simulink model "V0"  (R2026b)
settings: Solver=VariableStepAuto  MaxStep=1e-3
undefined symbols (not defined in the file): X, Y, Z
libraries: sm_lib x30, nesl_utility x7
settings Model: Creator=Alex  LastModifiedBy=Providenta
settings RTWCC: GPUComputeCapability=5.0
settings SimscapeCC: SimscapeUseEnergyAccounting=off
settings ExplorerConfigSet: InternalSimMechanicsExplorerSettings=|
  | <ExplorerConfiguration>
  | 
  |   <canonicalview>default</canonicalview>
  | 
  |   <TilePanel>
  |     <TileInfo>
  |       <Tiles Columns="1" Count="1" Height="506" Rows="1" Width="626">
  |         <Row Weight="1"/>
  |         <Column Weight="1"/>
  |         <Tile Height="1" Width="1" X="0" Y="0"/>
  |       </Tiles>
  |     </TileInfo>
  |     <SceneInfo>
  |       <SceneViewer>
  |         <IsThisViewStd>
  |           <IsStandardView>off</IsStandardView>
  |           <StandardViewName>Front</StandardViewName>
  |         </IsThisViewStd>
  |         <BGColor>
  |           <R>1</R>
  |           <G>1</G>
  |           <B>1</B>
  |           <A>1</A>
  |         </BGColor>
  |         <Camera>
  |           <DoPerspective>off</DoPerspective>
  |           <Position>
  |             <X>-1.2632471406802588</X>
  |             <Y>1.7763638648148106</Y>
  |             <Z>1.5649874221387672</Z>
  |           </Position>
  |           <Center>
  |             <X>0.25024160266871465</X>
  |             <Y>0.26287512146583708</Y>
  |             <Z>0.051498678789793695</Z>
  |           </Center>
  |           <Up>
  |             <X>0.40824829046386307</X>
  |             <Y>-0.40824829046386307</Y>
  |             <Z>0.81649658092772615</Z>
  |           </Up>
  |           <XLim>0.3536848912827506</XLim>
  |           <YLim>0.3536848912827506</YLim>
  |           <ViewLimDist>0.01</ViewLimDist>
  |         </Camera>
  |       </SceneViewer>
  |     </SceneInfo>
  |   </TilePanel>
  | 
  |   <MechEditorPanel>
  |     <GfxPanelCameraMap/>
  |     <Cameras/>
  |     <VideoCreator>
  |       <IncludeTiles>All</IncludeTiles>
  |       <IncludeTime>on</IncludeTime>
  |       <IncludeWorldFrame>off</IncludeWorldFrame>
  |       <PlaybackSpeedRatio>1</PlaybackSpeedRatio>
  |       <FrameRate>30</FrameRate>
  |       <FrameSize>auto</FrameSize>
  |       <VideoFormat>UncompressedAVI</VideoFormat>
  |     </VideoCreator>
  |   </MechEditorPanel>
  | 
  |   <PlaybackSettings>
  |     <PlaybackSpeedFactor>2</PlaybackSpeedFactor>
  |   </PlaybackSettings>
  | 
  | </ExplorerConfiguration>

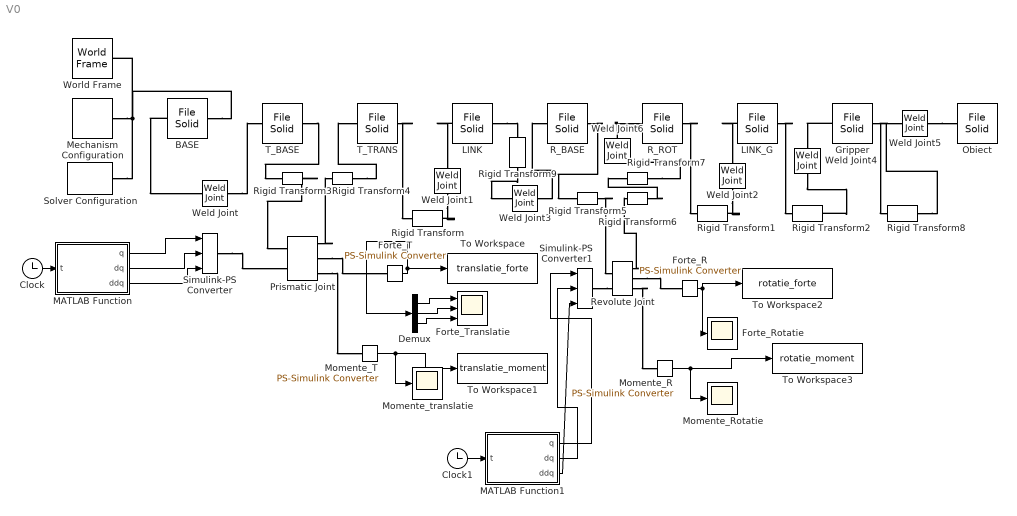
== system V0 ==
  BASE : sm_lib/Body Elements/File Solid  ExtGeomFileName=C:\Users\Georgian\Documents\PROBO\Objects\Links\Base.CATPart  UnitType=FromFile  ExtGeomFileUnits=m  StepReaderType=HEX  ExportConvexHullGeometry=off  InertiaType=CalculateFromGeometry  BasedOnType=DensityFromFile  Density=1000  DensityUnits=kg/m^3  Mass=1  MassUnits=kg  CenterOfMass=[0 0 0]  CenterOfMassUnits=m  MomentsOfInertia=[1 1 1]  MomentsOfInertiaUnits=kg*m^2  ProductsOfInertia=[0 0 0]  ProductsOfInertiaUnits=kg*m^2  GraphicType=FromGeometry  MarkerShape=Sphere  MarkerSize=10  GraphicVisPropType=SimpleVisualProperties  GraphicDiffuseColor=[0.5 0.5 0.5]  GraphicOpacity=1  GraphicSpecularColor=[0.5 0.5 0.5 1.0]  GraphicAmbientColor=[0.15 0.15 0.15 1.0]  GraphicEmissiveColor=[0.0 0.0 0.0 1.0]  GraphicShininess=75  DoExposeReferenceFrame=on  SerializedFrames=<Frames><Frame><Id>Frame1</Id><Value><Name>Main_LINK</Name><Origin><Source>GeometricFeature</Source><FeatureName>planar surface 2</FeatureName></Origin><PrimaryAxis><DefinedDirection>+Y</DefinedDirection><Source>ReferenceFrame</Source><SourceDirection>-Y</SourceDirection><FeatureName></FeatureName></PrimaryAxis><SecondaryAxis><DefinedDirection>+X</DefinedDirection><Source>ReferenceFrame</Source><SourceDirection>+X</SourceDirection><FeatureName></FeatureName></SecondaryAxis></Value></Frame></Frames>
  Clock : Clock
  Clock1 : Clock
  Demux : Demux  Outputs=3
  Forte_R : nesl_utility/PS-Simulink Converter  PhysicalDomain=network_engine_domain  SubClassName=ps_output  LeftPortType=input  RightPortType=output  PseudoPeriodic=off  Frequencies=[]  VectorFormat=inherit  Unit=inherit  AffineConversion=off
  Forte_Rotatie : Scope
      settings: ActiveDisplayYMinimum=-165.96901704363273  ActiveDisplayYMaximum=591.60143737609849  DataLoggingVariableName=ScopeData2
  Forte_T : nesl_utility/PS-Simulink Converter  PhysicalDomain=network_engine_domain  SubClassName=ps_output  LeftPortType=input  RightPortType=output  PseudoPeriodic=off  Frequencies=[]  VectorFormat=inherit  Unit=inherit  AffineConversion=off
  Forte_Translatie : Scope  NumInputPorts=3
      settings: ActiveDisplayYMinimum=-453.2641950281286  ActiveDisplayYMaximum=842.77836421107531
  Gripper : sm_lib/Body Elements/File Solid  ExtGeomFileName=C:\Users\Georgian\Documents\PROBO\Objects\Subansamblu_Gripper_fara_ob.stp  UnitType=FromFile  ExtGeomFileUnits=m  StepReaderType=HEX  ExportConvexHullGeometry=off  InertiaType=Custom  BasedOnType=DensityFromFile  Density=1000  DensityUnits=kg/m^3  Mass=4.055  MassUnits=kg  CenterOfMass=[0.0003906 79.531 -4.359]  CenterOfMassUnits=mm  MomentsOfInertia=[0.036 0.027 0.02]  MomentsOfInertiaUnits=kg*m^2  ProductsOfInertia=[-1.269e-5 -0.002 -1.039e-8]  ProductsOfInertiaUnits=kg*m^2  GraphicType=FromGeometry  MarkerShape=Sphere  MarkerSize=10  GraphicVisPropType=SimpleVisualProperties  GraphicDiffuseColor=[0.5 0.5 0.5]  GraphicOpacity=1  GraphicSpecularColor=[0.5 0.5 0.5 1.0]  GraphicAmbientColor=[0.15 0.15 0.15 1.0]  GraphicEmissiveColor=[0.0 0.0 0.0 1.0]  GraphicShininess=75  DoExposeReferenceFrame=off  SerializedFrames=<Frames><Frame><Id>Frame1</Id><Value><Name>R</Name><Origin><Source>GeometricFeature</Source><FeatureName>planar surface 481</FeatureName></Origin><PrimaryAxis><DefinedDirection>+Y</DefinedDirection><Source>ReferenceFrame</Source><SourceDirection>+Y</SourceDirection><FeatureName></FeatureName></PrimaryAxis><SecondaryAxis><DefinedDirection>+X</DefinedDirection><Source>ReferenceFrame</Source><SourceDirection>+X</SourceDirection><FeatureName></FeatureName></SecondaryAxis></Value></Frame><Frame><Id>Frame2</Id><Value><Name>F</Name><Origin><Source>GeometricFeature</Source><FeatureName>planar surface 1100</FeatureName></Origin><PrimaryAxis><DefinedDirection>+Z</DefinedDirection><Source>ReferenceFrame</Source><SourceDirection>+Z</SourceDirection><FeatureName></FeatureName></PrimaryAxis><SecondaryAxis><DefinedDirection>+X</DefinedDirection><Source>ReferenceFrame</Source><SourceDirection>+X</SourceDirection><FeatureName></FeatureName></SecondaryAxis></Value></Frame></Frames>
  LINK : sm_lib/Body Elements/File Solid  ExtGeomFileName=C:\Users\Georgian\Documents\PROBO\Objects\Links\Cot.CATPart  UnitType=FromFile  ExtGeomFileUnits=m  StepReaderType=HEX  ExportConvexHullGeometry=off  InertiaType=CalculateFromGeometry  BasedOnType=DensityFromFile  Density=1000  DensityUnits=kg/m^3  Mass=1  MassUnits=kg  CenterOfMass=[0 0 0]  CenterOfMassUnits=m  MomentsOfInertia=[1 1 1]  MomentsOfInertiaUnits=kg*m^2  ProductsOfInertia=[0 0 0]  ProductsOfInertiaUnits=kg*m^2  GraphicType=FromGeometry  MarkerShape=Sphere  MarkerSize=10  GraphicVisPropType=SimpleVisualProperties  GraphicDiffuseColor=[0.5 0.5 0.5]  GraphicOpacity=1  GraphicSpecularColor=[0.5 0.5 0.5 1.0]  GraphicAmbientColor=[0.15 0.15 0.15 1.0]  GraphicEmissiveColor=[0.0 0.0 0.0 1.0]  GraphicShininess=75  DoExposeReferenceFrame=off  SerializedFrames=|
      | <Frames>
      | 
      |   <Frame>
      |     <Id>Frame1</Id>
      |     <Value>
      |       <Name>F1</Name>
      |       <Origin>
      |         <Source>GeometricFeature</Source>
      |         <FeatureName>planar surface 2</FeatureName>
      |       </Origin>
      |       <PrimaryAxis>
      |         <DefinedDirection>+Z</DefinedDirection>
      |         <Source>ReferenceFrame</Source>
      |         <SourceDirection>+Z</SourceDirection>
      |         <FeatureName></FeatureName>
      |       </PrimaryAxis>
      |       <SecondaryAxis>
      |         <DefinedDirection>+X</DefinedDirection>
      |         <Source>ReferenceFrame</Source>
      |         <SourceDirection>+X</SourceDirection>
      |         <FeatureName></FeatureName>
      |       </SecondaryAxis>
      |     </Value>
      |   </Frame>
      | 
      |   <Frame>
      |     <Id>Frame2</Id>
      |     <Value>
      |       <Name>F2</Name>
      |       <Origin>
      |         <Source>GeometricFeature</Source>
      |         <FeatureName>planar surface 4</FeatureName>
      |       </Origin>
      |       <PrimaryAxis>
      |         <DefinedDirection>+Z</DefinedDirection>
      |         <Source>ReferenceFrame</Source>
      |         <SourceDirection>+Z</SourceDirection>
      |         <FeatureName></FeatureName>
      |       </PrimaryAxis>
      |       <SecondaryAxis>
      |         <DefinedDirection>+X</DefinedDirection>
      |         <Source>ReferenceFrame</Source>
      |         <SourceDirection>+X</SourceDirection>
      |         <FeatureName></FeatureName>
      |       </SecondaryAxis>
      |     </Value>
      |   </Frame>
      | 
      | </Frames>
  LINK_G : sm_lib/Body Elements/File Solid  ExtGeomFileName=C:\Users\Georgian\Documents\PROBO\Objects\LINK_MODUL2\LINK_G_MR.step  UnitType=FromFile  ExtGeomFileUnits=m  StepReaderType=HEX  ExportConvexHullGeometry=off  InertiaType=Custom  BasedOnType=DensityFromFile  Density=1000  DensityUnits=kg/m^3  Mass=1.753  MassUnits=kg  CenterOfMass=[0 -38.58 157.13]  CenterOfMassUnits=mm  MomentsOfInertia=[0.011 0.013 0.001]  MomentsOfInertiaUnits=kg*m^2  ProductsOfInertia=[0 0 0.001]  ProductsOfInertiaUnits=kg*m^2  GraphicType=FromGeometry  MarkerShape=Sphere  MarkerSize=10  GraphicVisPropType=SimpleVisualProperties  GraphicDiffuseColor=[0.5 0.5 0.5]  GraphicOpacity=1  GraphicSpecularColor=[0.5 0.5 0.5 1.0]  GraphicAmbientColor=[0.15 0.15 0.15 1.0]  GraphicEmissiveColor=[0.0 0.0 0.0 1.0]  GraphicShininess=75  DoExposeReferenceFrame=off  SerializedFrames=<Frames><Frame><Id>Frame1</Id><Value><Name>R</Name><Origin><Source>GeometricFeature</Source><FeatureName>planar surface 1</FeatureName></Origin><PrimaryAxis><DefinedDirection>+Z</DefinedDirection><Source>ReferenceFrame</Source><SourceDirection>+Z</SourceDirection><FeatureName></FeatureName></PrimaryAxis><SecondaryAxis><DefinedDirection>+X</DefinedDirection><Source>ReferenceFrame</Source><SourceDirection>+X</SourceDirection><FeatureName></FeatureName></SecondaryAxis></Value></Frame><Frame><Id>Frame2</Id><Value><Name>F</Name><Origin><Source>GeometricFeature</Source><FeatureName>planar surface 41</FeatureName></Origin><PrimaryAxis><DefinedDirection>+Y</DefinedDirection><Source>ReferenceFrame</Source><SourceDirection>+Y</SourceDirection><FeatureName></FeatureName></PrimaryAxis><SecondaryAxis><DefinedDirection>+X</DefinedDirection><Source>ReferenceFrame</Source><SourceDirection>+X</SourceDirection><FeatureName></FeatureName></SecondaryAxis></Value></Frame></Frames>
  MATLAB Function : MATLAB Function  TreatAsAtomicUnit=on
  MATLAB Function1 : MATLAB Function  TreatAsAtomicUnit=on
  Mechanism Configuration : sm_lib/Utilities/Mechanism Configuration  UniformGravity=Constant  GravityVector=[0 0 -9.80665]  GravityVectorUnits=m/s^2  LinearizationDelta=0.001  JointModeTransitionNonlinearIterations=2
  Momente_R : nesl_utility/PS-Simulink Converter  PhysicalDomain=network_engine_domain  SubClassName=ps_output  LeftPortType=input  RightPortType=output  PseudoPeriodic=off  Frequencies=[]  VectorFormat=inherit  Unit=inherit  AffineConversion=off
  Momente_Rotatie : Scope
      settings: ActiveDisplayYMinimum=-181.02759056182146  ActiveDisplayYMaximum=207.23761817348006  DataLoggingVariableName=ScopeData3
  Momente_T : nesl_utility/PS-Simulink Converter  PhysicalDomain=network_engine_domain  SubClassName=ps_output  LeftPortType=input  RightPortType=output  PseudoPeriodic=off  Frequencies=[]  VectorFormat=inherit  Unit=inherit  AffineConversion=off
  Momente_translatie : Scope
      settings: ActiveDisplayYMinimum=-251.95677444746502  ActiveDisplayYMaximum=342.42507637342931
  Obiect : sm_lib/Body Elements/File Solid  ExtGeomFileName=C:\Users\Georgian\Documents\PROBO\Objects\Paralelipiped.CATPart  UnitType=FromFile  ExtGeomFileUnits=m  StepReaderType=HEX  ExportConvexHullGeometry=off  InertiaType=Custom  BasedOnType=DensityFromFile  Density=1000  DensityUnits=kg/m^3  Mass=32.54  MassUnits=kg  CenterOfMass=[0 0 115]  CenterOfMassUnits=mm  MomentsOfInertia=[0.171 0.231 0.115]  MomentsOfInertiaUnits=kg*m^2  ProductsOfInertia=[0 0 0]  ProductsOfInertiaUnits=kg*m^2  GraphicType=FromGeometry  MarkerShape=Sphere  MarkerSize=10  GraphicVisPropType=SimpleVisualProperties  GraphicDiffuseColor=[0.5 0.5 0.5]  GraphicOpacity=1  GraphicSpecularColor=[0.5 0.5 0.5 1.0]  GraphicAmbientColor=[0.15 0.15 0.15 1.0]  GraphicEmissiveColor=[0.0 0.0 0.0 1.0]  GraphicShininess=75  DoExposeReferenceFrame=off  SerializedFrames=<Frames><Frame><Id>Frame1</Id><Value><Name>R</Name><Origin><Source>GeometricFeature</Source><FeatureName>planar surface 4</FeatureName></Origin><PrimaryAxis><DefinedDirection>+Z</DefinedDirection><Source>ReferenceFrame</Source><SourceDirection>+Z</SourceDirection><FeatureName></FeatureName></PrimaryAxis><SecondaryAxis><DefinedDirection>+X</DefinedDirection><Source>ReferenceFrame</Source><SourceDirection>+X</SourceDirection><FeatureName></FeatureName></SecondaryAxis></Value></Frame></Frames>
  Prismatic Joint : sm_lib/Joints/Prismatic Joint  JointMode=Normal  CompositeWrenchDir=FollowerOnBase  CompositeWrenchFrame=BaseFrame  SenseConstraintForce=off  SenseConstraintTorque=off  SenseTotalForce=on  SenseTotalTorque=on  PositionTargetSpecify=off  PositionTargetPriority=High  PositionTargetValue=0  PositionTargetValueUnits=m  VelocityTargetSpecify=off  VelocityTargetPriority=High  VelocityTargetValue=0  VelocityTargetValueUnits=m/s  EquilibriumPosition=0  EquilibriumPositionUnits=m  SpringStiffness=0  SpringStiffnessUnits=N/m  DampingCoefficient=0  DampingCoefficientUnits=N/(m/s)  LowerLimitSpecify=off  LowerLimitBound=-1  LowerLimitBoundUnits=m  LowerLimitStiffness=1e6  LowerLimitStiffnessUnits=N/m  LowerLimitDamping=1e3  LowerLimitDampingUnits=N/(m/s)  LowerLimitTransitionRegionWidth=1e-4  LowerLimitTransitionRegionWidthUnits=m  UpperLimitSpecify=off  UpperLimitBound=1  UpperLimitBoundUnits=m  UpperLimitStiffness=1e6  UpperLimitStiffnessUnits=N/m  UpperLimitDamping=1e3  UpperLimitDampingUnits=N/(m/s)  UpperLimitTransitionRegionWidth=1e-4  UpperLimitTransitionRegionWidthUnits=m  TorqueActuationMode=ComputedTorque  MotionActuationMode=InputMotion  SensePosition=off  SenseVelocity=off  SenseAcceleration=off  SenseTorqueForce=off  SenseLowerLimitTorqueForce=off  SenseUpperLimitTorqueForce=off
  R_BASE : sm_lib/Body Elements/File Solid  ExtGeomFileName=C:\Users\Georgian\Documents\PROBO\Objects\MODUL 2\R_STABIL\R_STABIL.stp  UnitType=FromFile  ExtGeomFileUnits=m  StepReaderType=HEX  ExportConvexHullGeometry=off  InertiaType=Custom  BasedOnType=DensityFromFile  Density=1000  DensityUnits=kg/m^3  Mass=4.576  MassUnits=kg  CenterOfMass=[0 0 -42.1]  CenterOfMassUnits=mm  MomentsOfInertia=[3.787e-2 3.787e-2 8.59e-3]  MomentsOfInertiaUnits=kg*m^2  ProductsOfInertia=[0 0 0]  ProductsOfInertiaUnits=kg*m^2  GraphicType=FromGeometry  MarkerShape=Sphere  MarkerSize=10  GraphicVisPropType=SimpleVisualProperties  GraphicDiffuseColor=[0.5 0.5 0.5]  GraphicOpacity=1  GraphicSpecularColor=[0.5 0.5 0.5 1.0]  GraphicAmbientColor=[0.15 0.15 0.15 1.0]  GraphicEmissiveColor=[0.0 0.0 0.0 1.0]  GraphicShininess=75  DoExposeReferenceFrame=off  SerializedFrames=<Frames><Frame><Id>Frame1</Id><Value><Name>R</Name><Origin><Source>GeometricFeature</Source><FeatureName>planar surface 141</FeatureName></Origin><PrimaryAxis><DefinedDirection>+Z</DefinedDirection><Source>ReferenceFrame</Source><SourceDirection>+Z</SourceDirection><FeatureName></FeatureName></PrimaryAxis><SecondaryAxis><DefinedDirection>+X</DefinedDirection><Source>ReferenceFrame</Source><SourceDirection>+X</SourceDirection><FeatureName></FeatureName></SecondaryAxis></Value></Frame><Frame><Id>Frame2</Id><Value><Name>F2</Name><Origin><Source>GeometricFeature</Source><FeatureName>planar surface 199</FeatureName></Origin><PrimaryAxis><DefinedDirection>+Z</DefinedDirection><Source>ReferenceFrame</Source><SourceDirection>+Z</SourceDirection><FeatureName></FeatureName></PrimaryAxis><SecondaryAxis><DefinedDirection>+X</DefinedDirection><Source>ReferenceFrame</Source><SourceDirection>+X</SourceDirection><FeatureName></FeatureName></SecondaryAxis></Value></Frame></Frames>
  R_ROT : sm_lib/Body Elements/File Solid  ExtGeomFileName=C:\Users\Georgian\Documents\PROBO\Objects\MODUL 2\R_MOBIL\R_MOBIL.stp  UnitType=FromFile  ExtGeomFileUnits=m  StepReaderType=HEX  ExportConvexHullGeometry=off  InertiaType=Custom  BasedOnType=DensityFromFile  Density=1000  DensityUnits=kg/m^3  Mass=0.3668  MassUnits=kg  CenterOfMass=[0 0 56.03]  CenterOfMassUnits=mm  MomentsOfInertia=[1.086e-4 1.069e-4 1.647e-4]  MomentsOfInertiaUnits=kg*m^2  ProductsOfInertia=[0 0 -2.83e-7]  ProductsOfInertiaUnits=kg*m^2  GraphicType=FromGeometry  MarkerShape=Sphere  MarkerSize=10  GraphicVisPropType=SimpleVisualProperties  GraphicDiffuseColor=[0.5 0.5 0.5]  GraphicOpacity=1  GraphicSpecularColor=[0.5 0.5 0.5 1.0]  GraphicAmbientColor=[0.15 0.15 0.15 1.0]  GraphicEmissiveColor=[0.0 0.0 0.0 1.0]  GraphicShininess=75  DoExposeReferenceFrame=off  SerializedFrames=<Frames><Frame><Id>Frame1</Id><Value><Name>R</Name><Origin><Source>GeometricFeature</Source><FeatureName>planar surface 20</FeatureName></Origin><PrimaryAxis><DefinedDirection>+Y</DefinedDirection><Source>ReferenceFrame</Source><SourceDirection>+Y</SourceDirection><FeatureName></FeatureName></PrimaryAxis><SecondaryAxis><DefinedDirection>+X</DefinedDirection><Source>ReferenceFrame</Source><SourceDirection>+X</SourceDirection><FeatureName></FeatureName></SecondaryAxis></Value></Frame><Frame><Id>Frame2</Id><Value><Name>F</Name><Origin><Source>GeometricFeature</Source><FeatureName>planar surface 22</FeatureName></Origin><PrimaryAxis><DefinedDirection>+Z</DefinedDirection><Source>ReferenceFrame</Source><SourceDirection>+Z</SourceDirection><FeatureName></FeatureName></PrimaryAxis><SecondaryAxis><DefinedDirection>+X</DefinedDirection><Source>ReferenceFrame</Source><SourceDirection>+X</SourceDirection><FeatureName></FeatureName></SecondaryAxis></Value></Frame></Frames>
  Revolute Joint : sm_lib/Joints/Revolute Joint  JointMode=Normal  CompositeWrenchDir=FollowerOnBase  CompositeWrenchFrame=BaseFrame  SenseConstraintForce=off  SenseConstraintTorque=off  SenseTotalForce=on  SenseTotalTorque=on  PositionTargetSpecify=off  PositionTargetPriority=High  PositionTargetValue=0  PositionTargetValueUnits=deg  VelocityTargetSpecify=off  VelocityTargetPriority=High  VelocityTargetValue=0  VelocityTargetValueUnits=deg/s  EquilibriumPosition=0  EquilibriumPositionUnits=deg  SpringStiffness=0  SpringStiffnessUnits=N*m/deg  DampingCoefficient=0  DampingCoefficientUnits=N*m/(deg/s)  LowerLimitSpecify=off  LowerLimitBound=-90  LowerLimitBoundUnits=deg  LowerLimitStiffness=1e4  LowerLimitStiffnessUnits=N*m/deg  LowerLimitDamping=10  LowerLimitDampingUnits=N*m/(deg/s)  LowerLimitTransitionRegionWidth=0.1  LowerLimitTransitionRegionWidthUnits=deg  UpperLimitSpecify=off  UpperLimitBound=90  UpperLimitBoundUnits=deg  UpperLimitStiffness=1e4  UpperLimitStiffnessUnits=N*m/deg  UpperLimitDamping=10  UpperLimitDampingUnits=N*m/(deg/s)  UpperLimitTransitionRegionWidth=0.1  UpperLimitTransitionRegionWidthUnits=deg  TorqueActuationMode=ComputedTorque  MotionActuationMode=InputMotion  SensePosition=off  SenseVelocity=off  SenseAcceleration=off  SenseTorqueForce=off  SenseLowerLimitTorqueForce=off  SenseUpperLimitTorqueForce=off
  Rigid Transform : sm_lib/Frames and Transforms/Rigid Transform  RotationMethod=RotationSequence  FollAlignAxisA=+X  BaseAlignAxisA=+Y  FollAlignAxisB=+Y  BaseAlignAxisB=+Z  RotationStandardAxis=+Y  RotationAngle=90  RotationAngleUnits=deg  RotationArbitraryAxis=[0 0 1]  RotationSequenceAxes=FollowerAxes  RotationSequence=YZX  RotationSequenceAngles=[90 180 0]  RotationSequenceAnglesUnits=deg  RotationMatrix=[1 0 0;0 1 0;0 0 1]  Quaternion=[1 0 0 0]  TranslationMethod=None  TranslationCartesianOffset=[0 0 0]  TranslationCartesianOffsetUnits=m  TranslationStandardAxis=+Z  TranslationStandardOffset=0  TranslationStandardOffsetUnits=m  TranslationROffset=0  TranslationROffsetUnits=m  TranslationThetaOffset=0  TranslationThetaOffsetUnits=deg  TranslationZOffset=0  TranslationZOffsetUnits=m
  Rigid Transform1 : sm_lib/Frames and Transforms/Rigid Transform  RotationMethod=RotationSequence  FollAlignAxisA=+X  BaseAlignAxisA=+Y  FollAlignAxisB=+Y  BaseAlignAxisB=+Z  RotationStandardAxis=+Z  RotationAngle=180  RotationAngleUnits=deg  RotationArbitraryAxis=[0 0 1]  RotationSequenceAxes=FollowerAxes  RotationSequence=ZXY  RotationSequenceAngles=[180 0 0]  RotationSequenceAnglesUnits=deg  RotationMatrix=[1 0 0;0 1 0;0 0 1]  Quaternion=[1 0 0 0]  TranslationMethod=Cartesian  TranslationCartesianOffset=[0 20 0]  TranslationCartesianOffsetUnits=mm  TranslationStandardAxis=+Z  TranslationStandardOffset=0  TranslationStandardOffsetUnits=m  TranslationROffset=0  TranslationROffsetUnits=m  TranslationThetaOffset=0  TranslationThetaOffsetUnits=deg  TranslationZOffset=0  TranslationZOffsetUnits=m
  Rigid Transform2 : sm_lib/Frames and Transforms/Rigid Transform  RotationMethod=RotationSequence  FollAlignAxisA=+X  BaseAlignAxisA=+Y  FollAlignAxisB=+Y  BaseAlignAxisB=+Z  RotationStandardAxis=+Z  RotationAngle=180  RotationAngleUnits=deg  RotationArbitraryAxis=[0 0 1]  RotationSequenceAxes=FollowerAxes  RotationSequence=ZXY  RotationSequenceAngles=[0 180 180]  RotationSequenceAnglesUnits=deg  RotationMatrix=[1 0 0;0 1 0;0 0 1]  Quaternion=[1 0 0 0]  TranslationMethod=Cartesian  TranslationCartesianOffset=[0 -60 +200]  TranslationCartesianOffsetUnits=mm  TranslationStandardAxis=+Z  TranslationStandardOffset=0  TranslationStandardOffsetUnits=m  TranslationROffset=0  TranslationROffsetUnits=m  TranslationThetaOffset=0  TranslationThetaOffsetUnits=deg  TranslationZOffset=0  TranslationZOffsetUnits=m
  Rigid Transform3 : sm_lib/Frames and Transforms/Rigid Transform  RotationMethod=RotationSequence  FollAlignAxisA=+X  BaseAlignAxisA=+Y  FollAlignAxisB=+Y  BaseAlignAxisB=+Z  RotationStandardAxis=+X  RotationAngle=-90  RotationAngleUnits=deg  RotationArbitraryAxis=[0 0 1]  RotationSequenceAxes=FollowerAxes  RotationSequence=YZX  RotationSequenceAngles=[-180 0 -90]  RotationSequenceAnglesUnits=deg  RotationMatrix=[1 0 0;0 1 0;0 0 1]  Quaternion=[1 0 0 0]  TranslationMethod=None  TranslationCartesianOffset=[-325 -20 0]  TranslationCartesianOffsetUnits=mm  TranslationStandardAxis=+X  TranslationStandardOffset=-325/2  TranslationStandardOffsetUnits=mm  TranslationROffset=0  TranslationROffsetUnits=m  TranslationThetaOffset=0  TranslationThetaOffsetUnits=deg  TranslationZOffset=0  TranslationZOffsetUnits=m
  Rigid Transform4 : sm_lib/Frames and Transforms/Rigid Transform  RotationMethod=RotationSequence  FollAlignAxisA=+X  BaseAlignAxisA=+Y  FollAlignAxisB=+Y  BaseAlignAxisB=+Z  RotationStandardAxis=+X  RotationAngle=+90  RotationAngleUnits=deg  RotationArbitraryAxis=[0 0 1]  RotationSequenceAxes=FollowerAxes  RotationSequence=YZX  RotationSequenceAngles=[180 0 -90]  RotationSequenceAnglesUnits=deg  RotationMatrix=[1 0 0;0 1 0;0 0 1]  Quaternion=[1 0 0 0]  TranslationMethod=None  TranslationCartesianOffset=[-325 -20 0]  TranslationCartesianOffsetUnits=mm  TranslationStandardAxis=+Y  TranslationStandardOffset=-325/2  TranslationStandardOffsetUnits=mm  TranslationROffset=0  TranslationROffsetUnits=m  TranslationThetaOffset=0  TranslationThetaOffsetUnits=deg  TranslationZOffset=0  TranslationZOffsetUnits=m
  Rigid Transform5 : sm_lib/Frames and Transforms/Rigid Transform  RotationMethod=StandardAxis  FollAlignAxisA=+X  BaseAlignAxisA=+Y  FollAlignAxisB=+Y  BaseAlignAxisB=+Z  RotationStandardAxis=+Z  RotationAngle=0  RotationAngleUnits=deg  RotationArbitraryAxis=[0 0 1]  RotationSequenceAxes=FollowerAxes  RotationSequence=YZX  RotationSequenceAngles=[90 180 0]  RotationSequenceAnglesUnits=deg  RotationMatrix=[1 0 0;0 1 0;0 0 1]  Quaternion=[1 0 0 0]  TranslationMethod=None  TranslationCartesianOffset=[0 0 0]  TranslationCartesianOffsetUnits=m  TranslationStandardAxis=+Z  TranslationStandardOffset=0  TranslationStandardOffsetUnits=m  TranslationROffset=0  TranslationROffsetUnits=m  TranslationThetaOffset=0  TranslationThetaOffsetUnits=deg  TranslationZOffset=0  TranslationZOffsetUnits=m
  Rigid Transform6 : sm_lib/Frames and Transforms/Rigid Transform  RotationMethod=StandardAxis  FollAlignAxisA=+X  BaseAlignAxisA=+Y  FollAlignAxisB=+Y  BaseAlignAxisB=+Z  RotationStandardAxis=+Z  RotationAngle=0  RotationAngleUnits=deg  RotationArbitraryAxis=[0 0 1]  RotationSequenceAxes=FollowerAxes  RotationSequence=YZX  RotationSequenceAngles=[90 180 0]  RotationSequenceAnglesUnits=deg  RotationMatrix=[1 0 0;0 1 0;0 0 1]  Quaternion=[1 0 0 0]  TranslationMethod=None  TranslationCartesianOffset=[0 0 0]  TranslationCartesianOffsetUnits=m  TranslationStandardAxis=+Z  TranslationStandardOffset=0  TranslationStandardOffsetUnits=m  TranslationROffset=0  TranslationROffsetUnits=m  TranslationThetaOffset=0  TranslationThetaOffsetUnits=deg  TranslationZOffset=0  TranslationZOffsetUnits=m
  Rigid Transform7 : sm_lib/Frames and Transforms/Rigid Transform  RotationMethod=RotationSequence  FollAlignAxisA=+X  BaseAlignAxisA=+Y  FollAlignAxisB=+Y  BaseAlignAxisB=+Z  RotationStandardAxis=+Z  RotationAngle=+180  RotationAngleUnits=deg  RotationArbitraryAxis=[0 0 1]  RotationSequenceAxes=FollowerAxes  RotationSequence=XYZ  RotationSequenceAngles=[180 180 0]  RotationSequenceAnglesUnits=deg  RotationMatrix=[1 0 0;0 1 0;0 0 1]  Quaternion=[1 0 0 0]  TranslationMethod=None  TranslationCartesianOffset=[0 0 0]  TranslationCartesianOffsetUnits=m  TranslationStandardAxis=+Z  TranslationStandardOffset=0  TranslationStandardOffsetUnits=m  TranslationROffset=0  TranslationROffsetUnits=m  TranslationThetaOffset=0  TranslationThetaOffsetUnits=deg  TranslationZOffset=0  TranslationZOffsetUnits=m
  Rigid Transform8 : sm_lib/Frames and Transforms/Rigid Transform  RotationMethod=RotationSequence  FollAlignAxisA=+X  BaseAlignAxisA=+Y  FollAlignAxisB=+Y  BaseAlignAxisB=+Z  RotationStandardAxis=+Z  RotationAngle=180  RotationAngleUnits=deg  RotationArbitraryAxis=[0 0 1]  RotationSequenceAxes=FollowerAxes  RotationSequence=ZXY  RotationSequenceAngles=[90 0 0]  RotationSequenceAnglesUnits=deg  RotationMatrix=[1 0 0;0 1 0;0 0 1]  Quaternion=[1 0 0 0]  TranslationMethod=Cartesian  TranslationCartesianOffset=[-30 70 -115]  TranslationCartesianOffsetUnits=mm  TranslationStandardAxis=+Z  TranslationStandardOffset=0  TranslationStandardOffsetUnits=m  TranslationROffset=0  TranslationROffsetUnits=m  TranslationThetaOffset=0  TranslationThetaOffsetUnits=deg  TranslationZOffset=0  TranslationZOffsetUnits=m
  Rigid Transform9 : sm_lib/Frames and Transforms/Rigid Transform  RotationMethod=RotationSequence  FollAlignAxisA=+X  BaseAlignAxisA=+Y  FollAlignAxisB=+Y  BaseAlignAxisB=+Z  RotationStandardAxis=+Y  RotationAngle=90  RotationAngleUnits=deg  RotationArbitraryAxis=[0 0 1]  RotationSequenceAxes=FollowerAxes  RotationSequence=YZX  RotationSequenceAngles=[0 0 -90]  RotationSequenceAnglesUnits=deg  RotationMatrix=[1 0 0;0 1 0;0 0 1]  Quaternion=[1 0 0 0]  TranslationMethod=None  TranslationCartesianOffset=[0 0 0]  TranslationCartesianOffsetUnits=m  TranslationStandardAxis=+Z  TranslationStandardOffset=0  TranslationStandardOffsetUnits=m  TranslationROffset=0  TranslationROffsetUnits=m  TranslationThetaOffset=0  TranslationThetaOffsetUnits=deg  TranslationZOffset=0  TranslationZOffsetUnits=m
  Simulink-PS Converter : nesl_utility/Simulink-PS Converter  PhysicalDomain=network_engine_domain  SubClassName=ps_input  LeftPortType=input  RightPortType=output  PseudoPeriodic=off  Frequencies=[]  NoiseDistribution=none  NoiseParameters=[]  Unit=1  AffineConversion=off  FilteringAndDerivatives=provide  SimscapeFilterOrder=1  InputFilterTimeConstant=0.001  UdotUserProvided=2
  Simulink-PS Converter1 : nesl_utility/Simulink-PS Converter  PhysicalDomain=network_engine_domain  SubClassName=ps_input  LeftPortType=input  RightPortType=output  PseudoPeriodic=off  Frequencies=[]  NoiseDistribution=none  NoiseParameters=[]  Unit=1  AffineConversion=off  FilteringAndDerivatives=provide  SimscapeFilterOrder=1  InputFilterTimeConstant=0.001  UdotUserProvided=2
  Solver Configuration : nesl_utility/Solver Configuration  PhysicalDomain=network_engine_domain  SubClassName=solver  LeftPortType=input  RightPortType=generic  Tones=[]  Harmonics=[]  SimulateNoise=off  Profile=off  UseLocalSampling=off  EnableSwitchedLinearOptims=on  FrequencyDomain=off  UseCCode=off  RelTol=0.001  AbsTol=0.001  MinStep=1e-09  ToWorkspace=off  RevertToSquareIcSolve=off  NumHomotopyIterations=100  PhasorMode=off  PhasorModeNumHarmonics=1  ConsistencySolver=NEWTON_XTOL_AFTER_FTOL  CanonicalOrdering=UNORDERED  OptimizeIntermediates=UNOPTIMIZED  MulticoreSolverChoice=BACKWARD_EULER  IndexReductionMethod=DerivativeReplacement  DoDC=off  ResidualTolerance=1e-09  ConsistencyTolSource=GLOBAL  ConsistencyAbsTol=0.001  ConsistencyRelTol=0.001  ConsistencyTolFactor=0.001  UseLocalSolver=off  LocalSolverChoice=NE_BACKWARD_EULER_ADVANCER  ResolveIndetEquations=on  FunctionEvalNumThread=1  LocalSolverSampleTime=0.001  DoFixedCost=off  MaxNonlinIter=3  MaxModeIter=2  ComputeImpulses=off  ImpulseIterations=2  LinearAlgebra=auto  LinearAlgebraNumThread=0  EquationFormulation=NE_TIME_EF  DelaysMemoryBudget=1024  AutomaticFiltering=on  FilteringTimeConstant=0.001  PartitionStorageMethod=AS_NEEDED  PartitionMemoryBudget=1024  PartitionMethod=BALANCED  MultibodyUseLocalSolver=off  MultibodyLocalSolverChoice=ODE1  MultibodyLocalSolverSampleTime=0.001
  T_BASE : sm_lib/Body Elements/File Solid  ExtGeomFileName=C:\Users\Georgian\Documents\PROBO\Objects\Links\T\T_Prisma.CATPart  UnitType=FromFile  ExtGeomFileUnits=m  StepReaderType=HEX  ExportConvexHullGeometry=off  InertiaType=CalculateFromGeometry  BasedOnType=DensityFromFile  Density=1000  DensityUnits=kg/m^3  Mass=1  MassUnits=kg  CenterOfMass=[0 0 0]  CenterOfMassUnits=m  MomentsOfInertia=[1 1 1]  MomentsOfInertiaUnits=kg*m^2  ProductsOfInertia=[0 0 0]  ProductsOfInertiaUnits=kg*m^2  GraphicType=FromGeometry  MarkerShape=Sphere  MarkerSize=10  GraphicVisPropType=SimpleVisualProperties  GraphicDiffuseColor=[0.5 0.5 0.5]  GraphicOpacity=1  GraphicSpecularColor=[0.5 0.5 0.5 1.0]  GraphicAmbientColor=[0.15 0.15 0.15 1.0]  GraphicEmissiveColor=[0.0 0.0 0.0 1.0]  GraphicShininess=75  DoExposeReferenceFrame=off  SerializedFrames=|
      | <Frames>
      | 
      |   <Frame>
      |     <Id>Frame1</Id>
      |     <Value>
      |       <Name>R</Name>
      |       <Origin>
      |         <Source>ReferenceFrame</Source>
      |         <FeatureName></FeatureName>
      |       </Origin>
      |       <PrimaryAxis>
      |         <DefinedDirection>+Z</DefinedDirection>
      |         <Source>ReferenceFrame</Source>
      |         <SourceDirection>+Z</SourceDirection>
      |         <FeatureName></FeatureName>
      |       </PrimaryAxis>
      |       <SecondaryAxis>
      |         <DefinedDirection>+X</DefinedDirection>
      |         <Source>ReferenceFrame</Source>
      |         <SourceDirection>+X</SourceDirection>
      |         <FeatureName></FeatureName>
      |       </SecondaryAxis>
      |     </Value>
      |   </Frame>
      | 
      |   <Frame>
      |     <Id>Frame2</Id>
      |     <Value>
      |       <Name>F</Name>
      |       <Origin>
      |         <Source>GeometricFeature</Source>
      |         <FeatureName>planar surface 6</FeatureName>
      |       </Origin>
      |       <PrimaryAxis>
      |         <DefinedDirection>+Z</DefinedDirection>
      |         <Source>ReferenceFrame</Source>
      |         <SourceDirection>+Z</SourceDirection>
      |         <FeatureName></FeatureName>
      |       </PrimaryAxis>
      |       <SecondaryAxis>
      |         <DefinedDirection>+X</DefinedDirection>
      |         <Source>ReferenceFrame</Source>
      |         <SourceDirection>+X</SourceDirection>
      |         <FeatureName></FeatureName>
      |       </SecondaryAxis>
      |     </Value>
      |   </Frame>
      | 
      | </Frames>
  T_TRANS : sm_lib/Body Elements/File Solid  ExtGeomFileName=C:\Users\Georgian\Documents\PROBO\Objects\Links\T\T_Cil.CATPart  UnitType=FromFile  ExtGeomFileUnits=m  StepReaderType=HEX  ExportConvexHullGeometry=off  InertiaType=CalculateFromGeometry  BasedOnType=DensityFromFile  Density=1000  DensityUnits=kg/m^3  Mass=1  MassUnits=kg  CenterOfMass=[0 0 0]  CenterOfMassUnits=m  MomentsOfInertia=[1 1 1]  MomentsOfInertiaUnits=kg*m^2  ProductsOfInertia=[0 0 0]  ProductsOfInertiaUnits=kg*m^2  GraphicType=FromGeometry  MarkerShape=Sphere  MarkerSize=10  GraphicVisPropType=SimpleVisualProperties  GraphicDiffuseColor=[0.5 0.5 0.5]  GraphicOpacity=1  GraphicSpecularColor=[0.5 0.5 0.5 1.0]  GraphicAmbientColor=[0.15 0.15 0.15 1.0]  GraphicEmissiveColor=[0.0 0.0 0.0 1.0]  GraphicShininess=75  DoExposeReferenceFrame=off  SerializedFrames=|
      | <Frames>
      | 
      |   <Frame>
      |     <Id>Frame1</Id>
      |     <Value>
      |       <Name>R</Name>
      |       <Origin>
      |         <Source>GeometricFeature</Source>
      |         <FeatureName>planar surface 3</FeatureName>
      |       </Origin>
      |       <PrimaryAxis>
      |         <DefinedDirection>+Z</DefinedDirection>
      |         <Source>ReferenceFrame</Source>
      |         <SourceDirection>+Z</SourceDirection>
      |         <FeatureName></FeatureName>
      |       </PrimaryAxis>
      |       <SecondaryAxis>
      |         <DefinedDirection>+X</DefinedDirection>
      |         <Source>ReferenceFrame</Source>
      |         <SourceDirection>+X</SourceDirection>
      |         <FeatureName></FeatureName>
      |       </SecondaryAxis>
      |     </Value>
      |   </Frame>
      | 
      |   <Frame>
      |     <Id>Frame2</Id>
      |     <Value>
      |       <Name>F</Name>
      |       <Origin>
      |         <Source>GeometricFeature</Source>
      |         <FeatureName>planar surface 2</FeatureName>
      |       </Origin>
      |       <PrimaryAxis>
      |         <DefinedDirection>+Z</DefinedDirection>
      |         <Source>ReferenceFrame</Source>
      |         <SourceDirection>+Z</SourceDirection>
      |         <FeatureName></FeatureName>
      |       </PrimaryAxis>
      |       <SecondaryAxis>
      |         <DefinedDirection>+X</DefinedDirection>
      |         <Source>ReferenceFrame</Source>
      |         <SourceDirection>+X</SourceDirection>
      |         <FeatureName></FeatureName>
      |       </SecondaryAxis>
      |     </Value>
      |   </Frame>
      | 
      | </Frames>
  To Workspace : ToWorkspace  VariableName=translatie_forte  SaveFormat=Timeseries  SampleTime=-1
  To Workspace1 : ToWorkspace  VariableName=translatie_moment  SaveFormat=Timeseries  SampleTime=-1
  To Workspace2 : ToWorkspace  VariableName=rotatie_forte  SaveFormat=Timeseries  SampleTime=-1
  To Workspace3 : ToWorkspace  VariableName=rotatie_moment  SaveFormat=Timeseries  SampleTime=-1
  Weld Joint{,1..6} (7 alike) : sm_lib/Joints/Weld Joint  JointMode=Normal  CompositeWrenchDir=FollowerOnBase  CompositeWrenchFrame=BaseFrame  SenseConstraintForce=off  SenseConstraintTorque=off  SenseTotalForce=off  SenseTotalTorque=off
  World Frame : sm_lib/Frames and Transforms/World Frame
  wires:
  Forte_T/1 -> Demux/1, To Workspace/1
  Momente_T/1 -> To Workspace1/1, Momente_translatie/1
  Momente_R/1 -> To Workspace3/1, Momente_Rotatie/1
  Forte_R/1 -> Forte_Rotatie/1, To Workspace2/1
  Demux/1 -> Forte_Translatie/1
  Demux/2 -> Forte_Translatie/2
  Demux/3 -> Forte_Translatie/3
  Clock/1 -> MATLAB Function/1(t)
  Clock1/1 -> MATLAB Function1/1(t)
  MATLAB Function/1(q) -> Simulink-PS Converter/1
  MATLAB Function/2(dq) -> Simulink-PS Converter/2
  MATLAB Function/3(ddq) -> Simulink-PS Converter/3
  MATLAB Function1/1(q) -> Simulink-PS Converter1/1
  MATLAB Function1/2(dq) -> Simulink-PS Converter1/2
  MATLAB Function1/3(ddq) -> Simulink-PS Converter1/3
  connections:
  Mechanism Configuration/RConn1 -- BASE/RConn1 -- World Frame/RConn1 -- Solver Configuration/RConn1
  BASE/LConn1 -- Weld Joint/LConn1
  LINK_G/LConn1 -- Weld Joint2/LConn1
  LINK_G/RConn1 -- Rigid Transform2/LConn1
  Gripper/LConn1 -- Weld Joint4/LConn1
  Weld Joint/RConn1 -- T_BASE/LConn1
  T_TRANS/RConn1 -- Rigid Transform/LConn1
  LINK/LConn1 -- Weld Joint1/LConn1
  LINK/RConn1 -- Rigid Transform9/LConn1
  R_ROT/RConn1 -- Rigid Transform1/LConn1
  Prismatic Joint/RConn2 -- Forte_T/LConn1
  Prismatic Joint/RConn3 -- Momente_T/LConn1
  Revolute Joint/RConn2 -- Forte_R/LConn1
  Revolute Joint/RConn3 -- Momente_R/LConn1
  T_BASE/RConn1 -- Rigid Transform3/LConn1
  Rigid Transform3/RConn1 -- Prismatic Joint/LConn1
  Prismatic Joint/RConn1 -- Rigid Transform4/LConn1
  Rigid Transform4/RConn1 -- T_TRANS/LConn1
  R_BASE/RConn1 -- Rigid Transform5/LConn1
  Rigid Transform5/RConn1 -- Revolute Joint/LConn1
  Revolute Joint/RConn1 -- Rigid Transform6/LConn1
  Weld Joint3/RConn1 -- R_BASE/LConn1
  Rigid Transform6/RConn1 -- Rigid Transform7/LConn1
  Rigid Transform7/RConn1 -- Weld Joint6/RConn1
  Weld Joint1/RConn1 -- Rigid Transform/RConn1
  Weld Joint2/RConn1 -- Rigid Transform1/RConn1
  Weld Joint4/RConn1 -- Rigid Transform2/RConn1
  Weld Joint5/RConn1 -- Obiect/LConn1
  Gripper/RConn1 -- Rigid Transform8/LConn1
  Rigid Transform8/RConn1 -- Weld Joint5/LConn1
  Weld Joint6/LConn1 -- R_ROT/LConn1
  Simulink-PS Converter/RConn1 -- Prismatic Joint/LConn2
  Simulink-PS Converter1/RConn1 -- Revolute Joint/LConn2
  Rigid Transform9/RConn1 -- Weld Joint3/LConn1

== matlab function V0/MATLAB Function1 ==
  data: t input; q output; dq output; ddq output
function [q, dq, ddq] = profil_R(t)
% PROFIL TRAPEZOIDAL DE VITEZA CU COLTURI ROTUNJITE - CUPLA DE ROTATIE (R)
% Viteza si acceleratia MAXIME ale modulului.
% Secventa:  0 (mijloc) -> +L/2 -> -L/2 -> +L/2 -> -L/2 ...
%            (cu L = 300 grade: 0 -> +150 -> -150 -> +150 ...)
% Fiecare cursa: trapez de viteza cu colturi rotunjite (acceleratie sin^2):
%   aceeasi viteza maxima v si acceleratie maxima a, dar fara salturi.
% Iesiri: q [rad], dq [rad/s], ddq [rad/s^2]

q = 0; dq = 0; ddq = 0;          % initializare (necesar in Simulink)

% ---------------- LIMITELE MODULULUI DE ROTATIE ----------------
L_lim = 300;      % unghi maxim (cursa totala) [grade]
V_lim = 120;      % viteza unghiulara maxima [grade/s]
A_lim = 510;      % acceleratia unghiulara maxima [grade/s^2]
% ---------------- MISCAREA CERUTA ----------------
L      = 300;     % cursa totala [grade] -> de la -L/2 la +L/2 (negativ = intai spre minus)
V      = 120;     % viteza [grade/s]      (maxima)
A      = 510;     % acceleratie [grade/s^2] (maxima)
t_p    = 0;       % pauza la capete [s]
repeta = true;    % true = continua +150 <-> -150; false = se opreste la -150
% --------------------------------------------------

semn = sign(L);
L = min(abs(L), L_lim);
V = min(abs(V), V_lim);
A = min(abs(A), A_lim);

h = deg2rad(L) / 2;               % jumatate de cursa (150 grade) [rad]
v = deg2rad(V);
a = deg2rad(A);
t = max(t, 0);

if h > 0 && v > 0 && a > 0
    T1 = durata(h, v, a);         % 0 -> +h
    T2 = durata(2*h, v, a);       % +h -> -h (cursa intreaga)

    if t < T1                                     % 0 -> +150
        [q, dq, ddq] = cursa(t, h, v, a);
    elseif t < T1 + t_p                           % pauza la +150
        q = h;
    else
        tm = t - T1 - t_p;
        if ~repeta && tm >= T2                    % oprit la -150
            q = -h;
        else
            P = 2*(T2 + t_p);                     % perioada dus-intors
            k = mod(tm, P);
            if k < T2                             % +150 -> -150
                [s, ds, dds] = cursa(k, 2*h, v, a);
                q = h - s;  dq = -ds;  ddq = -dds;
            elseif k < T2 + t_p                   % pauza la -150
                q = -h;
            elseif k < 2*T2 + t_p                 % -150 -> +150
                [s, ds, dds] = cursa(k - T2 - t_p, 2*h, v, a);
                q = -h + s; dq = ds;   ddq = dds;
            else                                  % pauza la +150
                q = h;
            end
        end
    end
end

q = semn*q; dq = semn*dq; ddq = semn*ddq;
end

% ---------- durata unei curse de lungime D ----------
function T = durata(D, v, a)
T_a = 2*v / a;                    % accelerare cu profil sin^2 (medie a/2)
if D >= v * T_a
    T = D / v + T_a;              % cu palier de viteza constanta
else
    T = 2*sqrt(2*D / a);          % cursa scurta: fara palier
end
end

% ---------- o cursa 0 -> D, trapez cu colturi rotunjite (sin^2) ----------
% Viteza: urca de la 0 la v, palier v, coboara la 0 (forma de trapez),
% dar acceleratia nu mai sare in treapta: ddq = a*sin^2(pi*tau/T_a),
% porneste lin din 0, ajunge la a maxim si revine lin la 0.
% -> fortele si momentele (J*ddq + gravitatie + ...) sunt netede.
function [q, dq, ddq] = cursa(tt, D, v, a)
T_a = 2*v / a;
if D >= v * T_a
    t_c = D / v - T_a;
else
    T_a = sqrt(2*D / a); t_c = 0; v = a*T_a/2;
end
t_f = 2*T_a + t_c;
if tt < T_a                                   % Faza I: accelerare lina
    [q, dq, ddq] = rampa(tt, T_a, a);
elseif tt < T_a + t_c                         % Faza II: viteza constanta
    q = a*T_a^2/4 + v*(tt - T_a); dq = v; ddq = 0;
elseif tt < t_f                               % Faza III: franare lina
    [qr, dqr, ddqr] = rampa(t_f - tt, T_a, a);
    q = D - qr; dq = dqr; ddq = -ddqr;
else
    q = D; dq = 0; ddq = 0;
end
end

% ---------- rampa de accelerare sin^2, de la repaus ----------
function [q, dq, ddq] = rampa(tau, T_a, a)
w   = 2*pi / T_a;
ddq = a * sin(pi*tau/T_a)^2;
dq  = a * (tau/2 - sin(w*tau)/(2*w));
q   = a * (tau^2/4 + (cos(w*tau) - 1)/(2*w^2));
end

== matlab function V0/MATLAB Function ==
  data: t input; q output; dq output; ddq output
function [q, dq, ddq] = profil_T(t)
% PROFIL TRAPEZOIDAL DE VITEZA CU COLTURI ROTUNJITE - CUPLA DE TRANSLATIE (T)
% Viteza si acceleratia MAXIME ale modulului.
% Secventa: 0 -> L, apoi (daca repeta = true) L -> 0 -> L -> ...
% Iesiri: q [m], dq [m/s], ddq [m/s^2]

q = 0; dq = 0; ddq = 0;          % initializare (necesar in Simulink)

% ---------------- LIMITELE MODULULUI DE TRANSLATIE ----------------
L_lim = 325;      % cursa maxima [mm]
V_lim = 0.0007;      % viteza maxima [m/s]
A_lim = 0.0135;     % acceleratia maxima [m/s^2]
% ---------------- MISCAREA CERUTA ----------------
L      = -325;     % cursa [mm] (negativ = sens invers)
V      = 0.0007;     % viteza [m/s]      (maxima)
A      = 0.0135;    % acceleratie [m/s^2] (maxima)
t_p    = 0;       % pauza la capete [s]
repeta = false;   % false = o cursa si ramane la L; true = dus-intors continuu
% --------------------------------------------------

semn = sign(L);
L = min(abs(L), L_lim) / 1000;    % mm -> m (doar cursa!)
v = min(abs(V), V_lim);
a = min(abs(A), A_lim);
t = max(t, 0);

if L > 0 && v > 0 && a > 0
    T = durata(L, v, a);
    if ~repeta
        [q, dq, ddq] = cursa(min(t, T), L, v, a);
    else
        k = mod(t, 2*(T + t_p));
        if k < T                                  % 0 -> L
            [q, dq, ddq] = cursa(k, L, v, a);
        elseif k < T + t_p                        % pauza la L
            q = L;
        elseif k < 2*T + t_p                      % L -> 0
            [s, ds, dds] = cursa(k - T - t_p, L, v, a);
            q = L - s; dq = -ds; ddq = -dds;
        end                                       % altfel pauza la 0
    end
end

q = semn*q; dq = semn*dq; ddq = semn*ddq;
end

% ---------- durata unei curse de lungime D ----------
function T = durata(D, v, a)
T_a = 2*v / a;                    % accelerare cu profil sin^2 (medie a/2)
if D >= v * T_a
    T = D / v + T_a;              % cu palier de viteza constanta
else
    T = 2*sqrt(2*D / a);          % cursa scurta: fara palier
end
end

% ---------- o cursa 0 -> D, trapez cu colturi rotunjite (sin^2) ----------
% Viteza: urca de la 0 la v, palier v, coboara la 0 (forma de trapez),
% dar acceleratia nu mai sare in treapta: ddq = a*sin^2(pi*tau/T_a),
% porneste lin din 0, ajunge la a maxim si revine lin la 0.
% -> fortele si momentele (J*ddq + gravitatie + ...) sunt netede.
function [q, dq, ddq] = cursa(tt, D, v, a)
T_a = 2*v / a;
if D >= v * T_a
    t_c = D / v - T_a;
else
    T_a = sqrt(2*D / a); t_c = 0; v = a*T_a/2;
end
t_f = 2*T_a + t_c;
if tt < T_a                                   % Faza I: accelerare lina
    [q, dq, ddq] = rampa(tt, T_a, a);
elseif tt < T_a + t_c                         % Faza II: viteza constanta
    q = a*T_a^2/4 + v*(tt - T_a); dq = v; ddq = 0;
elseif tt < t_f                               % Faza III: franare lina
    [qr, dqr, ddqr] = rampa(t_f - tt, T_a, a);
    q = D - qr; dq = dqr; ddq = -ddqr;
else
    q = D; dq = 0; ddq = 0;
end
end

% ---------- rampa de accelerare sin^2, de la repaus ----------
function [q, dq, ddq] = rampa(tau, T_a, a)
w   = 2*pi / T_a;
ddq = a * sin(pi*tau/T_a)^2;
dq  = a * (tau/2 - sin(w*tau)/(2*w));
q   = a * (tau^2/4 + (cos(w*tau) - 1)/(2*w^2));
end
